simulink model "sensorExpoler"  (R2026a)
settings: Solver=FixedStepDiscrete  StopTime=30  FixedStep=0.001
PreLoadFcn:
  | t = pos_data.time;
  | p = pos_data.signals.values;
  | v = vel_data.signals.values;
  | 
  | T = table(t, p, v, 'VariableNames', {'Time_s', 'Position_rad', 'Velocity_rad_s'});
  | writetable(T, 'Lab1_3_Encoder_Data.csv');
  | disp('--- Export CSV Completed Automatically! ---');
InitFcn:
  | clear functions;
undefined symbols (not defined in the file or in its folder): Blocking, Non
libraries: amg_usbconverter_n_connect_lib x2
settings Model: Creator=pboon  LastModifiedBy=rosva

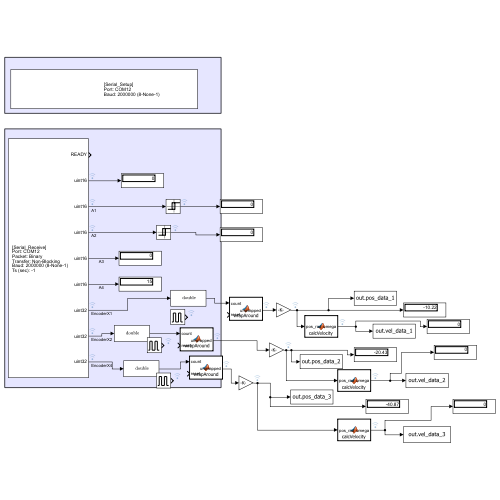
[thumbnail: Simulink's stored preview of the top-level diagram]
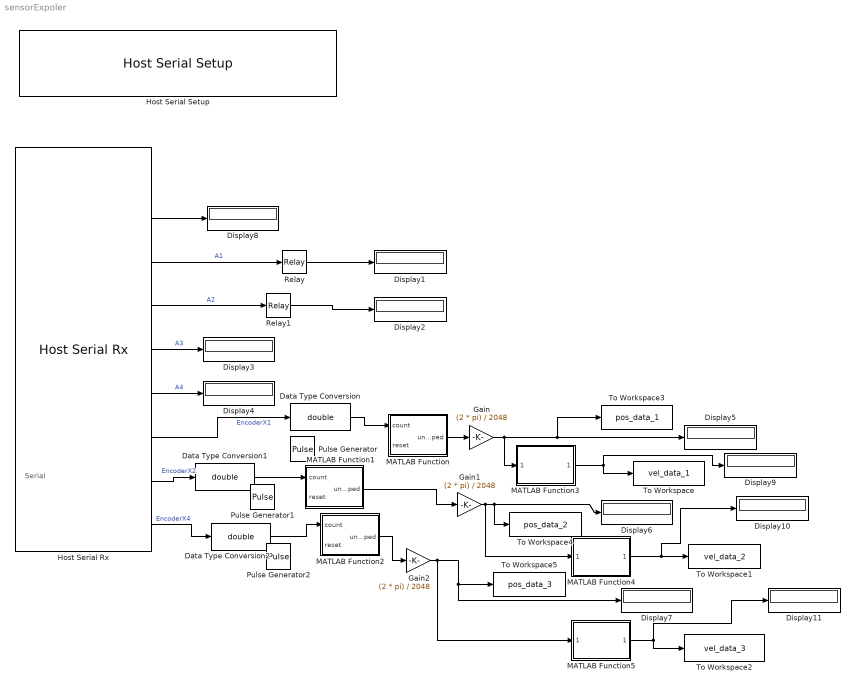
== system sensorExpoler ==
  note: Serial
  Data Type Conversion : DataTypeConversion  OutDataTypeStr=double  SaturateOnIntegerOverflow=off  RndMeth=Floor
  Data Type Conversion1 : DataTypeConversion  OutDataTypeStr=double  SaturateOnIntegerOverflow=off  RndMeth=Floor
  Data Type Conversion2 : DataTypeConversion  OutDataTypeStr=double  SaturateOnIntegerOverflow=off  RndMeth=Floor
  Display{1..11} (11 alike) : Display
  Gain : Gain  Gain=(2 * pi) / 2048
  Gain1 : Gain  Gain=(2 * pi) / 2048
  Gain2 : Gain  Gain=(2 * pi) / 2048
  Host Serial Rx : amg_usbconverter_n_connect_lib/Host Serial Rx  conf=rx  port=COM12  baudrate=2000000  databits=8  parity=None  stopbit=1  flowcontrol=None  transfer=Non-Blocking  timeout=5  packetmode=Binary  enableinitialvalues=off  initialvalues=[]  binheader='25'  binterminator='4E 4E'  porttype_double=0  porttype_single=0  porttype_int8=0  porttype_uint8=0  porttype_int16=0  porttype_uint16=5  porttype_int32=0  porttype_uint32=3  asciiformat='%d,%f'  rx_asciiterminator="CRLF (0x0D 0x0A - \"\\r\\n\")"  tx_asciiterminator="CRLF (0x0D 0x0A - \"\\r\\n\")"  sampletime=0.001  enablecustomportlabel=off  cinputportlabel=0  coutputportlabel=A  portpinstr=0  blockid=HostSerialRx  inputporttype=[]  inputportwidth=[]  inputportlabel={}  outputporttype=[3 5 5 5 5 5 7 7 7]  outputportwidth=[1 1 1 1 1 1 1 1 1]  outputportlabel={'READY','uint16','uint16','uint16','uint16','uint16','uint32','uint32','uint32'}  compat=0  optionstring=[]  autoport='COM12'
  Host Serial Setup : amg_usbconverter_n_connect_lib/Host Serial Setup  conf=setup  port=COM12  baudrate=2000000  databits=8  parity=None  stopbit=1  flowcontrol=None  transfer=Blocking  timeout=2  packetmode=Binary  initialvalues=[]  binheader='7E 7E'  binterminator='03 03'  porttype_double=0  porttype_single=1  porttype_int8=0  porttype_uint8=0  porttype_int16=0  porttype_uint16=0  porttype_int32=0  porttype_uint32=2  asciiformat='%d %u %x'  rx_asciiterminator="CRLF (0x0D 0x0A - \"\\r\\n\")"  tx_asciiterminator="CRLF (0x0D 0x0A - \"\\r\\n\")"  sampletime=-1  enablecustomportlabel=off  cinputportlabel=0  coutputportlabel=A  portpinstr=0  blockid=HostSerialSetup  inputporttype=[]  inputportwidth=[]  inputportlabel={}  outputporttype=[]  outputportwidth=[]  outputportlabel={}  compat=0  optionstring=[]  autoport='COM12'
  MATLAB Function : MATLAB Function  TreatAsAtomicUnit=on
  MATLAB Function1 : MATLAB Function  TreatAsAtomicUnit=on
  MATLAB Function2 : MATLAB Function  TreatAsAtomicUnit=on
  MATLAB Function3 : MATLAB Function  TreatAsAtomicUnit=on
  MATLAB Function4 : MATLAB Function  TreatAsAtomicUnit=on
  MATLAB Function5 : MATLAB Function  TreatAsAtomicUnit=on
  Pulse Generator : DiscretePulseGenerator  PulseType=Time based  Period=50  PulseWidth=10
  Pulse Generator1 : DiscretePulseGenerator  PulseType=Time based  Period=50  PulseWidth=10
  Pulse Generator2 : DiscretePulseGenerator  PulseType=Time based  Period=50  PulseWidth=10
  Relay : Relay  OnSwitchValue=2500  OffSwitchValue=1500
  Relay1 : Relay  OnSwitchValue=2500  OffSwitchValue=1500
  To Workspace : ToWorkspace  VariableName=vel_data_1  SaveFormat=Timeseries  SampleTime=-1
  To Workspace1 : ToWorkspace  VariableName=vel_data_2  SaveFormat=Timeseries  SampleTime=-1
  To Workspace2 : ToWorkspace  VariableName=vel_data_3  SaveFormat=Timeseries  SampleTime=-1
  To Workspace3 : ToWorkspace  VariableName=pos_data_1  SaveFormat=Timeseries  SampleTime=-1
  To Workspace4 : ToWorkspace  VariableName=pos_data_2  SaveFormat=Timeseries  SampleTime=-1
  To Workspace5 : ToWorkspace  VariableName=pos_data_3  SaveFormat=Timeseries  SampleTime=-1
  wires:
  Host Serial Rx/5 -> Display3/1  "A3"
  Host Serial Rx/6 -> Display4/1  "A4"
  Host Serial Rx/2 -> Display8/1
  Host Serial Rx/7 -> Data Type Conversion/1  "EncoderX1"
  Data Type Conversion/1 -> MATLAB Function/1(count)
  Host Serial Rx/8 -> Data Type Conversion1/1  "EncoderX2"
  Data Type Conversion1/1 -> MATLAB Function1/1(count)
  Host Serial Rx/9 -> Data Type Conversion2/1  "EncoderX4"
  Data Type Conversion2/1 -> MATLAB Function2/1(count)
  MATLAB Function/1(unwrapped) -> Gain/1
  MATLAB Function2/1(unwrapped) -> Gain2/1
  Gain2/1 -> MATLAB Function5/1(pos_rad), Display7/1, To Workspace5/1
  Host Serial Rx/3 -> Relay/1  "A1"
  Relay/1 -> Display1/1
  Host Serial Rx/4 -> Relay1/1  "A2"
  Relay1/1 -> Display2/1
  Gain/1 -> MATLAB Function3/1(pos_rad), To Workspace3/1, Display5/1
  MATLAB Function1/1(unwrapped) -> Gain1/1
  Gain1/1 -> MATLAB Function4/1(pos_rad), To Workspace4/1, Display6/1
  MATLAB Function3/1(omega) -> Display9/1, To Workspace/1
  MATLAB Function4/1(omega) -> Display10/1, To Workspace1/1
  MATLAB Function5/1(omega) -> Display11/1, To Workspace2/1

== matlab function sensorExpoler/MATLAB Function ==
  data: count input; unwrapped output; reset input
function unwrapped = wrapAround(count, reset)
    PERIOD = 65536; % Timer Period ของ STM32
    
    persistent prev_count accumulated_count
    
    if isempty(prev_count)
        prev_count = count;
        accumulated_count = 0;
    end

    % --- จังหวะ Auto Reset (เมื่อมีพัลส์ส่งมาจาก Pulse Generator) ---
    if reset > 0
        accumulated_count = 0;   % ล้างค่าตำแหน่งสะสมเป็น 0
        prev_count = count;      % ตั้งจุดอ้างอิงตำแหน่งนับใหม่
        unwrapped = 0;           % บังคับให้ส่งค่า 0 ออกทันที
    else
        % --- จังหวะคำนวณตำแหน่งปกติ ---
        diff = count - prev_count;
        
        % แก้ไข Timer Over/Underflow
        if diff > PERIOD / 2
            diff = diff - PERIOD;
        elseif diff < -PERIOD / 2
            diff = diff + PERIOD;
        end
        
        accumulated_count = accumulated_count + diff;
        prev_count = count;
        
        unwrapped = accumulated_count;
    end
end

== matlab function sensorExpoler/MATLAB Function2 ==
  data: count input; unwrapped output; reset input
function unwrapped = wrapAround(count, reset)
    PERIOD = 65536; % Timer Period ของ STM32
    
    persistent prev_count accumulated_count
    
    if isempty(prev_count)
        prev_count = count;
        accumulated_count = 0;
    end

    % --- จังหวะ Auto Reset (เมื่อมีพัลส์ส่งมาจาก Pulse Generator) ---
    if reset > 0
        accumulated_count = 0;   % ล้างค่าตำแหน่งสะสมเป็น 0
        prev_count = count;      % ตั้งจุดอ้างอิงตำแหน่งนับใหม่
        unwrapped = 0;           % บังคับให้ส่งค่า 0 ออกทันที
    else
        % --- จังหวะคำนวณตำแหน่งปกติ ---
        diff = count - prev_count;
        
        % แก้ไข Timer Over/Underflow
        if diff > PERIOD / 2
            diff = diff - PERIOD;
        elseif diff < -PERIOD / 2
            diff = diff + PERIOD;
        end
        
        accumulated_count = accumulated_count + diff;
        prev_count = count;
        
        unwrapped = accumulated_count;
    end
end

== matlab function sensorExpoler/MATLAB Function3 ==
  data: pos_rad input; omega output
function omega = calcVelocity(pos_rad)
    % 1. กำหนด Sample Time ของระบบ (ตั้งให้ตรงกับ Simulink เช่น 0.01 วินาที)
    Ts = 0.01; 
    
    % 2. ประกาศตัวแปรจดจำค่าตำแหน่งเดิมระหว่าง Sampling Loop
    persistent prev_pos
    
    % 3. กำหนดค่าเริ่มต้นเมื่อเริ่มรัน Simulation ครั้งแรก
    if isempty(prev_pos)
        prev_pos = pos_rad;
    end
    
    % 4. คำนวณความเร็วเชิงมุม omega = (theta_new - theta_old) / Ts
    omega = (pos_rad - prev_pos) / Ts;
    
    % 5. อัปเดตค่าตำแหน่งปัจจุบันไว้ใช้ในรอบถัดไป
    prev_pos = pos_rad;
end

== matlab function sensorExpoler/MATLAB Function4 ==
  data: pos_rad input; omega output
function omega = calcVelocity(pos_rad)
    % 1. กำหนด Sample Time ของระบบ (ตั้งให้ตรงกับ Simulink เช่น 0.01 วินาที)
    Ts = 0.01; 
    
    % 2. ประกาศตัวแปรจดจำค่าตำแหน่งเดิมระหว่าง Sampling Loop
    persistent prev_pos
    
    % 3. กำหนดค่าเริ่มต้นเมื่อเริ่มรัน Simulation ครั้งแรก
    if isempty(prev_pos)
        prev_pos = pos_rad;
    end
    
    % 4. คำนวณความเร็วเชิงมุม omega = (theta_new - theta_old) / Ts
    omega = (pos_rad - prev_pos) / Ts;
    
    % 5. อัปเดตค่าตำแหน่งปัจจุบันไว้ใช้ในรอบถัดไป
    prev_pos = pos_rad;
end

== matlab function sensorExpoler/MATLAB Function5 ==
  data: pos_rad input; omega output
function omega = calcVelocity(pos_rad)
    % 1. กำหนด Sample Time ของระบบ (ตั้งให้ตรงกับ Simulink เช่น 0.01 วินาที)
    Ts = 0.01; 
    
    % 2. ประกาศตัวแปรจดจำค่าตำแหน่งเดิมระหว่าง Sampling Loop
    persistent prev_pos
    
    % 3. กำหนดค่าเริ่มต้นเมื่อเริ่มรัน Simulation ครั้งแรก
    if isempty(prev_pos)
        prev_pos = pos_rad;
    end
    
    % 4. คำนวณความเร็วเชิงมุม omega = (theta_new - theta_old) / Ts
    omega = (pos_rad - prev_pos) / Ts;
    
    % 5. อัปเดตค่าตำแหน่งปัจจุบันไว้ใช้ในรอบถัดไป
    prev_pos = pos_rad;
end

== matlab function sensorExpoler/MATLAB Function1 ==
  data: count input; unwrapped output; reset input
function unwrapped = wrapAround(count, reset)
    PERIOD = 65536; % Timer Period ของ STM32
    
    persistent prev_count accumulated_count
    
    if isempty(prev_count)
        prev_count = count;
        accumulated_count = 0;
    end

    % --- จังหวะ Auto Reset (เมื่อมีพัลส์ส่งมาจาก Pulse Generator) ---
    if reset > 0
        accumulated_count = 0;   % ล้างค่าตำแหน่งสะสมเป็น 0
        prev_count = count;      % ตั้งจุดอ้างอิงตำแหน่งนับใหม่
        unwrapped = 0;           % บังคับให้ส่งค่า 0 ออกทันที
    else
        % --- จังหวะคำนวณตำแหน่งปกติ ---
        diff = count - prev_count;
        
        % แก้ไข Timer Over/Underflow
        if diff > PERIOD / 2
            diff = diff - PERIOD;
        elseif diff < -PERIOD / 2
            diff = diff + PERIOD;
        end
        
        accumulated_count = accumulated_count + diff;
        prev_count = count;
        
        unwrapped = accumulated_count;
    end
end
